simulink model "Kinematics_Front_Axle_"  (R2026a)
settings: Solver=ode23t  StopTime=2
undefined symbols (not defined in the file or in its folder): Camber_Clearance_Coeff, Jounce_Clearance_Coeff, Nominal_Clearance, Steer_Clearance_Coeff, X, Y, Z
libraries: sm_lib x4, nesl_utility x1
settings Model: Creator=Milán  LastModifiedBy=Milán

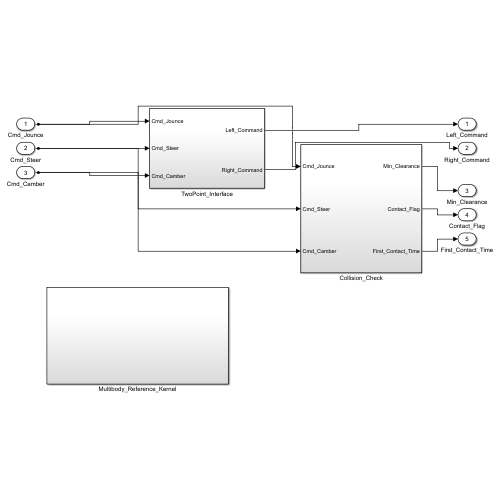
[thumbnail: Simulink's stored preview of the top-level diagram]
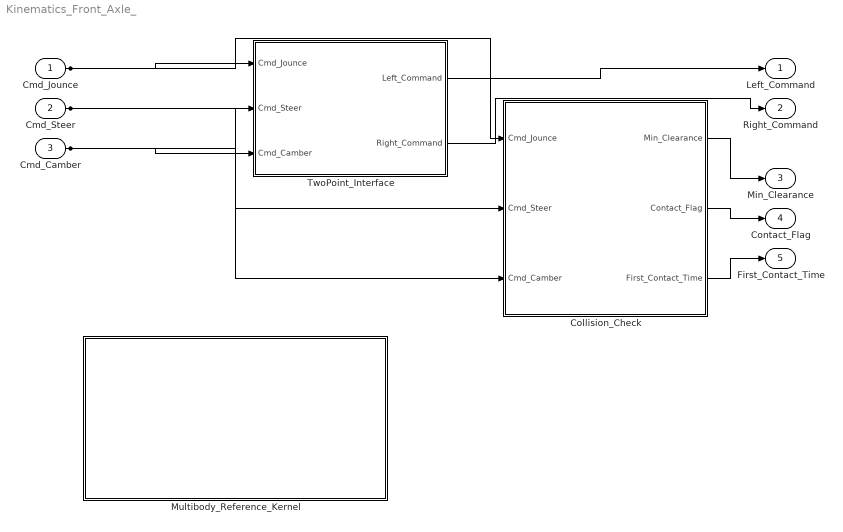
== system Kinematics_Front_Axle_ ==
  Cmd_Jounce : Inport
  Cmd_Steer : Inport  Port=2
  Cmd_Camber : Inport  Port=3
  Collision_Check : Subsystem
  Multibody_Reference_Kernel : Subsystem
  TwoPoint_Interface : Subsystem
  Left_Command : Outport
  Right_Command : Outport  Port=2
  Min_Clearance : Outport  Port=3
  Contact_Flag : Outport  Port=4
  First_Contact_Time : Outport  Port=5
  wires:
  Cmd_Jounce/1 -> TwoPoint_Interface/1(Cmd_Jounce), Collision_Check/1(Cmd_Jounce)
  Cmd_Steer/1 -> TwoPoint_Interface/2(Cmd_Steer), Collision_Check/2(Cmd_Steer)
  Cmd_Camber/1 -> TwoPoint_Interface/3(Cmd_Camber), Collision_Check/3(Cmd_Camber)
  TwoPoint_Interface/1(Left_Command) -> Left_Command/1
  TwoPoint_Interface/2(Right_Command) -> Right_Command/1
  Collision_Check/1(Min_Clearance) -> Min_Clearance/1
  Collision_Check/2(Contact_Flag) -> Contact_Flag/1
  Collision_Check/3(First_Contact_Time) -> First_Contact_Time/1

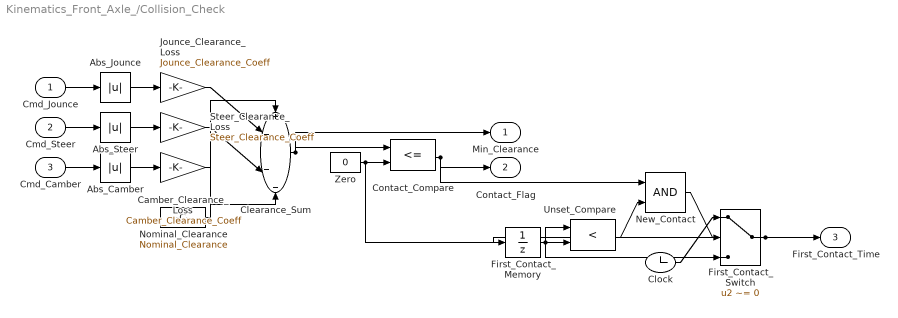
== system Kinematics_Front_Axle_/Collision_Check ==
  Cmd_Jounce : Inport
  Cmd_Steer : Inport  Port=2
  Cmd_Camber : Inport  Port=3
  Abs_Camber : Abs  SaturateOnIntegerOverflow=off
  Abs_Jounce : Abs  SaturateOnIntegerOverflow=off
  Abs_Steer : Abs  SaturateOnIntegerOverflow=off
  Camber_Clearance_Loss : Gain  Gain=Camber_Clearance_Coeff
  Clearance_Sum : Sum  Inputs=+---
  Clock : Clock
  Contact_Compare : RelationalOperator  Operator=<=  OutDataTypeStr=boolean  RndMeth=Simplest  InputSameDT=off
  First_Contact_Memory : UnitDelay  InitialCondition=-1  SampleTime=-1
  First_Contact_Switch : Switch  Criteria=u2 ~= 0  SaturateOnIntegerOverflow=off  InputSameDT=off
  Jounce_Clearance_Loss : Gain  Gain=Jounce_Clearance_Coeff
  New_Contact : Logic  AllPortsSameDT=off  OutDataTypeStr=boolean
  Nominal_Clearance : Constant  Value=Nominal_Clearance
  Steer_Clearance_Loss : Gain  Gain=Steer_Clearance_Coeff
  Unset_Compare : RelationalOperator  Operator=<  OutDataTypeStr=boolean  RndMeth=Simplest  InputSameDT=off
  Zero : Constant  Value=0
  Min_Clearance : Outport
  Contact_Flag : Outport  Port=2
  First_Contact_Time : Outport  Port=3
  wires:
  Cmd_Jounce/1 -> Abs_Jounce/1
  Cmd_Steer/1 -> Abs_Steer/1
  Cmd_Camber/1 -> Abs_Camber/1
  Abs_Jounce/1 -> Jounce_Clearance_Loss/1
  Abs_Steer/1 -> Steer_Clearance_Loss/1
  Abs_Camber/1 -> Camber_Clearance_Loss/1
  Nominal_Clearance/1 -> Clearance_Sum/1
  Jounce_Clearance_Loss/1 -> Clearance_Sum/2
  Steer_Clearance_Loss/1 -> Clearance_Sum/3
  Camber_Clearance_Loss/1 -> Clearance_Sum/4
  Clearance_Sum/1 -> Min_Clearance/1, Contact_Compare/1
  Zero/1 -> Contact_Compare/2, Unset_Compare/2
  Contact_Compare/1 -> Contact_Flag/1, New_Contact/1
  First_Contact_Memory/1 -> Unset_Compare/1, First_Contact_Switch/3
  Unset_Compare/1 -> New_Contact/2
  Clock/1 -> First_Contact_Switch/1
  New_Contact/1 -> First_Contact_Switch/2
  First_Contact_Switch/1 -> First_Contact_Memory/1, First_Contact_Time/1

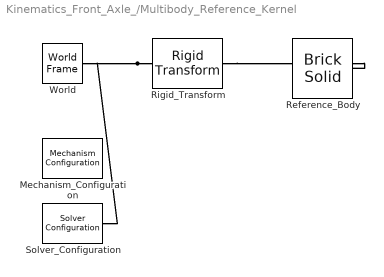
== system Kinematics_Front_Axle_/Multibody_Reference_Kernel ==
  Mechanism_Configuration : sm_lib/Utilities/Mechanism Configuration  UniformGravity=Constant  GravityVector=[0 0 -9.80665]  GravityVectorUnits=m/s^2  LinearizationDelta=0.001  JointModeTransitionNonlinearIterations=2
  Reference_Body : sm_lib/Body Elements/Brick Solid  BrickDimensions=[1 1 1]  BrickDimensionsUnits=m  ExportEntireGeometry=off  InertiaType=CalculateFromGeometry  BasedOnType=Density  Density=1000  DensityUnits=kg/m^3  Mass=1  MassUnits=kg  CenterOfMass=[0 0 0]  CenterOfMassUnits=m  MomentsOfInertia=[1 1 1]  MomentsOfInertiaUnits=kg*m^2  ProductsOfInertia=[0 0 0]  ProductsOfInertiaUnits=kg*m^2  GraphicType=FromGeometry  MarkerShape=Sphere  MarkerSize=10  GraphicVisPropType=SimpleVisualProperties  GraphicDiffuseColor=[0.5 0.5 0.5]  GraphicOpacity=1  GraphicSpecularColor=[0.5 0.5 0.5 1.0]  GraphicAmbientColor=[0.15 0.15 0.15 1.0]  GraphicEmissiveColor=[0.0 0.0 0.0 1.0]  GraphicShininess=75  DoExposeReferenceFrame=on  SerializedFrames=<Frames/>
  Rigid_Transform : sm_lib/Frames and Transforms/Rigid Transform  RotationMethod=None  FollAlignAxisA=+X  BaseAlignAxisA=+Y  FollAlignAxisB=+Y  BaseAlignAxisB=+Z  RotationStandardAxis=+Z  RotationAngle=0  RotationAngleUnits=deg  RotationArbitraryAxis=[0 0 1]  RotationSequenceAxes=FollowerAxes  RotationSequence=XYX  RotationSequenceAngles=[0 0 0]  RotationSequenceAnglesUnits=deg  RotationMatrix=[1 0 0;0 1 0;0 0 1]  Quaternion=[1 0 0 0]  TranslationMethod=None  TranslationCartesianOffset=[0 0 0]  TranslationCartesianOffsetUnits=m  TranslationStandardAxis=+Z  TranslationStandardOffset=0  TranslationStandardOffsetUnits=m  TranslationROffset=0  TranslationROffsetUnits=m  TranslationThetaOffset=0  TranslationThetaOffsetUnits=deg  TranslationZOffset=0  TranslationZOffsetUnits=m
  Solver_Configuration : nesl_utility/Solver Configuration  PhysicalDomain=network_engine_domain  SubClassName=solver  LeftPortType=input  RightPortType=generic  Tones=[]  Harmonics=[]  SimulateNoise=off  Profile=off  UseLocalSampling=off  EnableSwitchedLinearOptims=on  FrequencyDomain=off  UseCCode=off  RelTol=0.001  AbsTol=0.001  MinStep=1e-09  ToWorkspace=off  RevertToSquareIcSolve=off  NumHomotopyIterations=100  PhasorMode=off  PhasorModeNumHarmonics=1  ConsistencySolver=NEWTON_XTOL_AFTER_FTOL  CanonicalOrdering=CANONICAL  OptimizeIntermediates=OPTIMIZED  IndexReductionMethod=DerivativeReplacement  DoDC=off  ResidualTolerance=1e-09  ConsistencyTolSource=GLOBAL  ConsistencyAbsTol=0.001  ConsistencyRelTol=0.001  ConsistencyTolFactor=0.001  UseLocalSolver=off  LocalSolverChoice=NE_BACKWARD_EULER_ADVANCER  ResolveIndetEquations=on  FunctionEvalNumThread=1  LocalSolverSampleTime=0.001  DoFixedCost=off  MaxNonlinIter=3  MaxModeIter=2  ComputeImpulses=off  ImpulseIterations=2  LinearAlgebra=auto  LinearAlgebraNumThread=0  EquationFormulation=NE_TIME_EF  DelaysMemoryBudget=1024  AutomaticFiltering=on  FilteringTimeConstant=0.001  PartitionStorageMethod=AS_NEEDED  PartitionMemoryBudget=1024  PartitionMethod=ROBUST  MultibodyUseLocalSolver=off  MultibodyLocalSolverChoice=ODE1  MultibodyLocalSolverSampleTime=0.001
  World : sm_lib/Frames and Transforms/World Frame
  connections:
  Rigid_Transform/LConn1 -- World/RConn1 -- Solver_Configuration/RConn1
  Rigid_Transform/RConn1 -- Reference_Body/RConn1

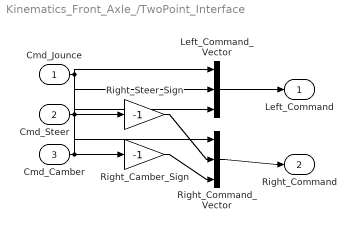
== system Kinematics_Front_Axle_/TwoPoint_Interface ==
  Cmd_Jounce : Inport
  Cmd_Steer : Inport  Port=2
  Cmd_Camber : Inport  Port=3
  Left_Command_Vector : Mux  Inputs=3
  Right_Camber_Sign : Gain  Gain=-1
  Right_Command_Vector : Mux  Inputs=3
  Right_Steer_Sign : Gain  Gain=-1
  Left_Command : Outport
  Right_Command : Outport  Port=2
  wires:
  Cmd_Jounce/1 -> Left_Command_Vector/1, Right_Command_Vector/1
  Cmd_Steer/1 -> Left_Command_Vector/2, Right_Steer_Sign/1
  Cmd_Camber/1 -> Left_Command_Vector/3, Right_Camber_Sign/1
  Right_Steer_Sign/1 -> Right_Command_Vector/2
  Right_Camber_Sign/1 -> Right_Command_Vector/3
  Left_Command_Vector/1 -> Left_Command/1
  Right_Command_Vector/1 -> Right_Command/1
